simulink model "ecu_gov"  (R2026a)
settings: Solver=FixedStepDiscrete  StopTime=10  FixedStep=0.001  SampleTimeConstraint=STIndependent
Description:
  | Speed governor. Source of truth for firmware/gen/gov; see model/README.md.
settings Model: Creator=jj1001000  LastModifiedBy=jj1001000
settings OptimizationCC: DefaultUnderspecifiedDataType=single
settings DebuggingCC: ParameterPrecisionLossMsg=none
settings HardwareCC: ProdLargestAtomicInteger=Long  ProdLargestAtomicFloat=Double  ProdHWDeviceType=ARM Compatible->ARM Cortex-M
settings RTWCC: SystemTargetFile=ert.tlc  GenCodeOnly=on  Description=Embedded Coder
settings ERTTargetCC: UtilityFuncGeneration=Shared location  IncludeMdlTerminateFcn=off  CodeInterfacePackaging=Reusable function  SupportNonFinite=off

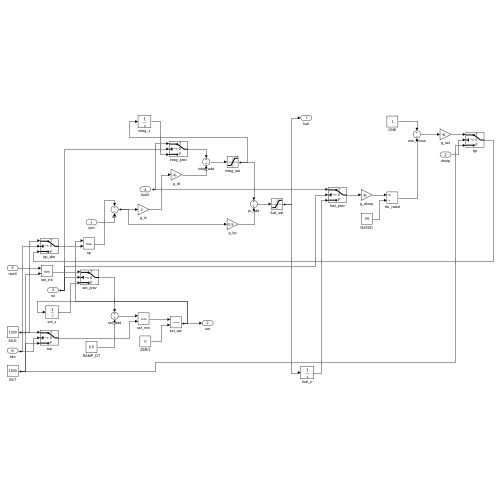
[thumbnail: Simulink's stored preview of the top-level diagram]
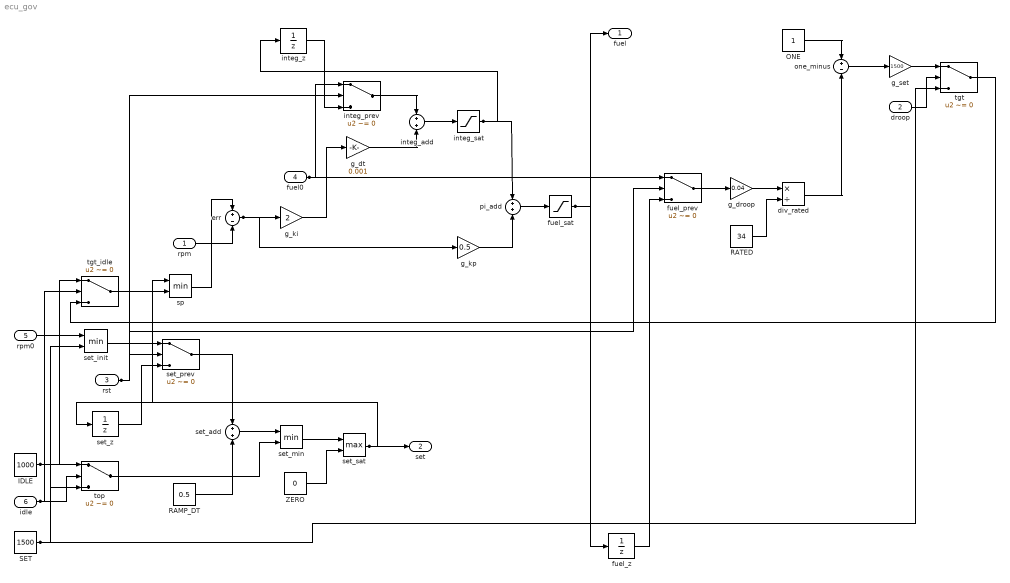
== system ecu_gov ==
  rpm : Inport  OutDataTypeStr=single
  droop : Inport  Port=2  OutDataTypeStr=uint8
  rst : Inport  Port=3  OutDataTypeStr=uint8
  fuel0 : Inport  Port=4  OutDataTypeStr=single
  rpm0 : Inport  Port=5  OutDataTypeStr=single
  idle : Inport  Port=6  OutDataTypeStr=uint8
  IDLE : Constant  Value=1000  OutDataTypeStr=single
  ONE : Constant  OutDataTypeStr=single
  RAMP_DT : Constant  Value=0.5  OutDataTypeStr=single
  RATED : Constant  Value=34  OutDataTypeStr=single
  SET : Constant  Value=1500  OutDataTypeStr=single
  ZERO : Constant  Value=0  OutDataTypeStr=single
  div_rated : Product  Inputs=*/
  err : Sum  Inputs=+-
  fuel_prev : Switch  Criteria=u2 ~= 0  SaturateOnIntegerOverflow=off  InputSameDT=off
  fuel_sat : Saturate  UpperLimit=45  LowerLimit=0
  fuel_z : UnitDelay  SampleTime=-1
  g_droop : Gain  Gain=0.04
  g_dt : Gain  Gain=0.001
  g_ki : Gain  Gain=2
  g_kp : Gain  Gain=0.5
  g_set : Gain  Gain=1500
  integ_add : Sum
  integ_prev : Switch  Criteria=u2 ~= 0  SaturateOnIntegerOverflow=off  InputSameDT=off
  integ_sat : Saturate  UpperLimit=45  LowerLimit=0
  integ_z : UnitDelay  SampleTime=-1
  one_minus : Sum  Inputs=+-
  pi_add : Sum
  set_add : Sum
  set_init : MinMax  Inputs=2
  set_min : MinMax  Inputs=2
  set_prev : Switch  Criteria=u2 ~= 0  SaturateOnIntegerOverflow=off  InputSameDT=off
  set_sat : MinMax  Function=max  Inputs=2
  set_z : UnitDelay  SampleTime=-1
  sp : MinMax  Inputs=2
  tgt : Switch  Criteria=u2 ~= 0  SaturateOnIntegerOverflow=off  InputSameDT=off
  tgt_idle : Switch  Criteria=u2 ~= 0  SaturateOnIntegerOverflow=off  InputSameDT=off
  top : Switch  Criteria=u2 ~= 0  SaturateOnIntegerOverflow=off  InputSameDT=off
  fuel : Outport  OutDataTypeStr=single
  set : Outport  Port=2  OutDataTypeStr=single
  wires:
  droop/1 -> tgt/2
  fuel0/1 -> fuel_prev/1, integ_prev/1
  rpm0/1 -> set_init/1
  rst/1 -> integ_prev/2, set_prev/2, fuel_prev/2
  set_prev/1 -> set_add/1
  IDLE/1 -> top/1, tgt_idle/1
  pi_add/1 -> fuel_sat/1
  idle/1 -> tgt_idle/2, top/2
  SET/1 -> top/3, set_init/2, tgt/3
  set_init/1 -> set_prev/1
  tgt_idle/1 -> sp/2
  set_z/1 -> set_prev/3
  top/1 -> set_min/2
  integ_prev/1 -> integ_add/1
  rpm/1 -> err/2
  sp/1 -> err/1
  set_add/1 -> set_min/1
  RAMP_DT/1 -> set_add/2
  err/1 -> g_kp/1, g_ki/1
  integ_z/1 -> integ_prev/3
  g_ki/1 -> g_dt/1
  fuel_sat/1 -> fuel/1, fuel_z/1
  set_min/1 -> set_sat/1
  ZERO/1 -> set_sat/2
  integ_add/1 -> integ_sat/1
  g_dt/1 -> integ_add/2
  set_sat/1 -> set_z/1, sp/1, set/1
  integ_sat/1 -> integ_z/1, pi_add/1
  g_kp/1 -> pi_add/2
  fuel_z/1 -> fuel_prev/3
  fuel_prev/1 -> g_droop/1
  ONE/1 -> one_minus/1
  g_droop/1 -> div_rated/1
  div_rated/1 -> one_minus/2
  RATED/1 -> div_rated/2
  tgt/1 -> tgt_idle/3
  one_minus/1 -> g_set/1
  g_set/1 -> tgt/1
